simulink model "phase6_regerative"  (R2025a)
settings: Solver=VariableStepAuto  StartTime=0.0  StopTime=5  RelTol=1e-3
model workspace (MAT data in the model file):
  AFE_id_ref_profile = timeseries
  AFE_id_ref_profile.Name = 'unnamed'
  AFE_id_ref_profile.DataInfo = tsdata.datametadata
  AFE_id_ref_profile.DataInfo.Interpolation = tsdata.interpolation
  AFE_id_ref_profile.DataInfo.Interpolation.Fhandle : function handle (value not decoded)
  AFE_id_ref_profile.DataInfo.Interpolation.Name = 'linear'
  AFE_id_ref_profile.TimeInfo = tsdata.timemetadata
  AFE_id_ref_profile.TimeInfo.Length = 6
  AFE_id_ref_profile.TimeInfo.DuplicateTimes = 0
  AFE_id_ref_profile.TimeInfo.Time_ = [0; 0.1; 2; 3; 3.1; 5]
  AFE_id_ref_profile.TimeInfo.Initialized = 1
  AFE_id_ref_profile.QualityInfo = tsdata.qualmetadata
  AFE_id_ref_profile.Data_ = [0.5; 0.5; 0.5; 0.5; -0.5; -0.5]
  G = 10
  Jeq = 0.8325
  Tgravity = 27.25
  eta = 0.9
  g = 9.81
  mc = 500
  mcw = 600
  mp = 200
  r = 0.25
  speed_cmd = timeseries
  speed_cmd.Name = 'unnamed'
  speed_cmd.DataInfo = tsdata.datametadata
  speed_cmd.DataInfo.Interpolation = tsdata.interpolation
  speed_cmd.DataInfo.Interpolation.Fhandle : function handle (value not decoded)
  speed_cmd.DataInfo.Interpolation.Name = 'linear'
  speed_cmd.TimeInfo = tsdata.timemetadata
  speed_cmd.TimeInfo.Length = 6
  speed_cmd.TimeInfo.DuplicateTimes = 0
  speed_cmd.TimeInfo.Time_ = [0; 0.1; 2; 3; 3.01; 5]
  speed_cmd.TimeInfo.Initialized = 1
  speed_cmd.QualityInfo = tsdata.qualmetadata
  speed_cmd.Data_ = [0; 0; 382; 382; 0; 0]
libraries: slpidlib x3, spsUniversalBridgeLib x2, eeGeneralControl x1, spsPLL3phLib x1, eePmsmFieldOrientedControl x1, spsPWMGenerator2LevelLib x1, spsPermanentMagnetSynchronousMachineLib x1, spsSeriesRLCBranchLib x1, spsThreePhaseSeriesRLCBranchLib x1, spsThreePhaseVIMeasurementLib x1, spsThreePhaseSourceLib x1, spsVoltageMeasurementLib x1
settings Model: Creator=kesav  LastModifiedBy=kesav
settings SolverCC: ZeroCrossAlgorithm=Adaptive

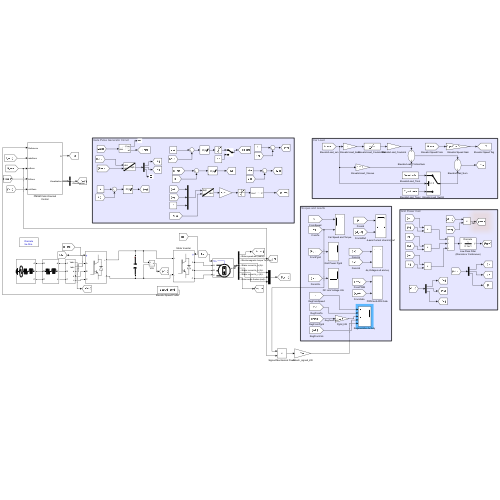
[thumbnail: Simulink's stored preview of the top-level diagram]
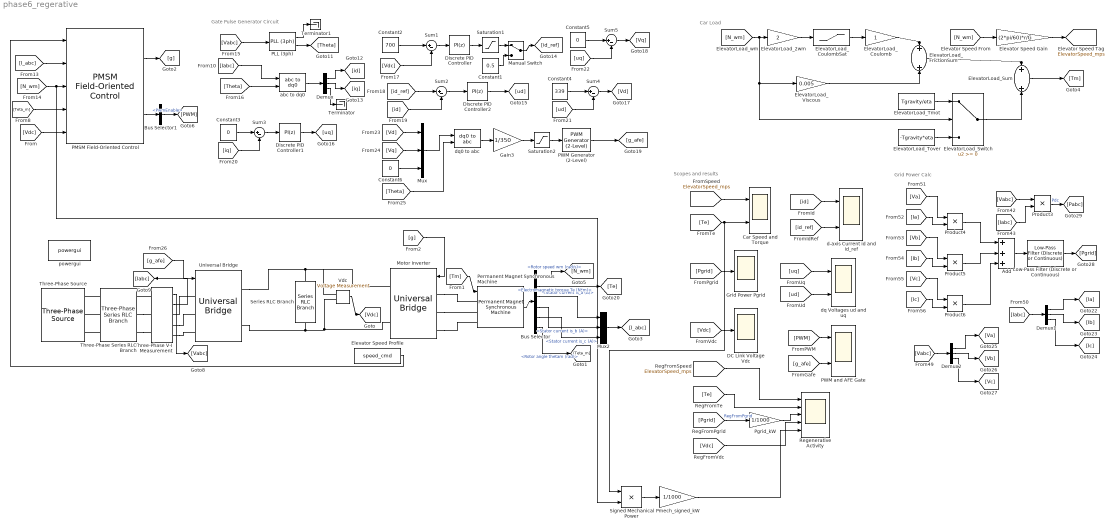
== system phase6_regerative ==
  note: Scopes and results
  note: Grid Power Calc
  note: Car Load
  note: Gate Pulse Generator Circuit
  Add : Sum  Inputs=+++
  Bus Selector : BusSelector  OutputSignals=Rotor speed wm (rad/s),Electromagnetic torque Te (N*m),Stator current is_a (A),Stator current is_b (A),Stator current is_c (A),Rotor angle thetam (rad)
  Bus Selector1 : BusSelector  OutputSignals=PwmEnable
  Car Speed and Torque : Scope  NumInputPorts=2
      settings: ActiveDisplayYMinimum=-0.021018648833083863  ActiveDisplayYMaximum=0.18916306327997173
  Constant1 : Constant  Value=0.5
  Constant2 : Constant  Value=700
  Constant3 : Constant  Value=0
  Constant4 : Constant  Value=339
  Constant5 : Constant  Value=0
  Constant6 : Constant  Value=0
  DC Link Voltage Vdc : Scope
      settings: DataLoggingVariableName=ScopeData2
  Demux : Demux  Outputs=3
  Demux1 : Demux  Outputs=3
  Demux2 : Demux  Outputs=3
  Discrete PID Controller : slpidlib/PID Controller  Controller=PI  Form=Parallel  TimeDomain=Discrete-time  UseExternalTs=off  SampleTime=1e-4  IntegratorMethod=Forward Euler  FilterMethod=Forward Euler  ControllerParametersSource=internal  P=0.5  I=15  UseKiTs=off  D=0  UseExternalDerivativeSource=off  N=100  UseFilter=on  TunerSelectOption=Transfer Function Based (PID Tuner App)  InitialConditionSource=internal  InitialConditionForIntegrator=0  InitialConditionForFilter=0  DifferentiatorICPrevScaledInput=0  ExternalReset=none  TrackingMode=off  Kt=1  LimitOutput=on  SatLimitsSource=internal  UpperSaturationLimit=20  LowerSaturationLimit=-20  LinearizeAsGain=off  AntiWindupMode=clamping  Kb=1  LimitIntegrator=off  UpperIntegratorSaturationLimit=inf  LowerIntegratorSaturationLimit=-inf  POutMin=[]  POutMax=[]  IOutMin=[]  IOutMax=[]  DOutMin=[]  DOutMax=[]  NOutMin=[]  NOutMax=[]  SumOutMin=[]  SumOutMax=[]  SaturationOutMin=[]  SaturationOutMax=[]  PParamMin=[]  PParamMax=[]  IParamMin=[]  IParamMax=[]  DParamMin=[]  DParamMax=[]  NParamMin=[]  NParamMax=[]  KbParamMin=[]  KbParamMax=[]  KtParamMin=[]  KtParamMax=[]  KbOutMin=[]  KbOutMax=[]  KtOutMin=[]  KtOutMax=[]  IntegratorOutMin=[]  IntegratorOutMax=[]  FilterOutMin=[]  FilterOutMax=[]  SumI1OutMin=[]  SumI1OutMax=[]  SumI2OutMin=[]  SumI2OutMax=[]  SumI3OutMin=[]  SumI3OutMax=[]  SumI4OutMin=[]  SumI4OutMax=[]  SumDOutMin=[]  SumDOutMax=[]  DifferentiatorOutMin=[]  DifferentiatorOutMax=[]  FilterDiffOutCoefMin=[]  FilterDiffOutCoefMax=[]  ReciprocalOutMin=[]  ReciprocalOutMax=[]  SumDenOutMin=[]  SumDenOutMax=[]  SumNumOutMin=[]  SumNumOutMax=[]  DivideOutMin=[]  DivideOutMax=[]  UdiffTsProdOutMin=[]  UdiffTsProdOutMax=[]  NTsProdOutMin=[]  NTsProdOutMax=[]  UintegralTsProdOutMin=[]  UintegralTsProdOutMax=[]  UngainTsProdOutMin=[]  UngainTsProdOutMax=[]  ClampingZeroOutDataTypeStr=Inherit: Inherit via back propagation  ClampingZeroOutMin=[]  ClampingZeroOutMax=[]  FilterDenConstantOutDataTypeStr=Inherit: Inherit via back propagation  FilterDenConstantOutMin=[]  FilterDenConstantOutMax=[]  PCopyOutDataTypeStr=Inherit: Inherit via back propagation  PCopyOutMin=[]  PCopyOutMax=[]  NCopyOutDataTypeStr=Inherit: Inherit via back propagation  NCopyOutMin=[]  NCopyOutMax=[]  IntegratorContinuousStateAttributes=''  IntegratorStateMustResolveToSignalObject=off  IntegratorRTWStateStorageClass=Auto  FilterContinuousStateAttributes=''  FilterStateMustResolveToSignalObject=off  FilterRTWStateStorageClass=Auto  ParallelPVariant=InternalParameters  IdealPVariant=Disabled  IVariant=InternalParameters  DVariant=Disabled  IntegratorVariant=Discrete  SatVariant=Enabled  AWVariant=DiscClampingParallel  PCopyVariant=Disabled  TRVariant=Disabled  FdbkBlocksVariant=Forward  IdealPFdbkVariant=Disabled  SatFdbkVariant=Disabled  DerivativeFilterVariant=Disabled  NVariant=Disabled  NCopyVariant=Disabled_SignalSpec  FilterICVariant=Disabled  IntegratorICVariant=InternalICs  ExternalResetVariant=Disabled  TRSumVariant=Passthrough  SumFdbkVariant=Disabled  SumVariant=Sum_PI  TsampFilterVariant=InternalTs  TsampNgainVariant=Passthrough  TsampIntegralVariant=Disabled_SignalSpec  ExternalSaturationOutDataTypeStr=Inherit: Same as second input  DerivativeSourceVariant=Disabled  PreIntVariant=InternalPreInt
      settings: LibrarySourceBlock=simulink/Discrete/Discrete PID Controller
  Discrete PID Controller1 : slpidlib/PID Controller  Controller=PI  Form=Parallel  TimeDomain=Discrete-time  UseExternalTs=off  SampleTime=5e-6  IntegratorMethod=Forward Euler  FilterMethod=Forward Euler  ControllerParametersSource=internal  P=15  I=30  UseKiTs=off  D=0  UseExternalDerivativeSource=off  N=100  UseFilter=on  TunerSelectOption=Transfer Function Based (PID Tuner App)  InitialConditionSource=internal  InitialConditionForIntegrator=0  InitialConditionForFilter=0  DifferentiatorICPrevScaledInput=0  ExternalReset=none  TrackingMode=off  Kt=1  LimitOutput=on  SatLimitsSource=internal  UpperSaturationLimit=350  LowerSaturationLimit=-350  LinearizeAsGain=off  AntiWindupMode=clamping  Kb=1  LimitIntegrator=off  UpperIntegratorSaturationLimit=inf  LowerIntegratorSaturationLimit=-inf  POutMin=[]  POutMax=[]  IOutMin=[]  IOutMax=[]  DOutMin=[]  DOutMax=[]  NOutMin=[]  NOutMax=[]  SumOutMin=[]  SumOutMax=[]  SaturationOutMin=[]  SaturationOutMax=[]  PParamMin=[]  PParamMax=[]  IParamMin=[]  IParamMax=[]  DParamMin=[]  DParamMax=[]  NParamMin=[]  NParamMax=[]  KbParamMin=[]  KbParamMax=[]  KtParamMin=[]  KtParamMax=[]  KbOutMin=[]  KbOutMax=[]  KtOutMin=[]  KtOutMax=[]  IntegratorOutMin=[]  IntegratorOutMax=[]  FilterOutMin=[]  FilterOutMax=[]  SumI1OutMin=[]  SumI1OutMax=[]  SumI2OutMin=[]  SumI2OutMax=[]  SumI3OutMin=[]  SumI3OutMax=[]  SumI4OutMin=[]  SumI4OutMax=[]  SumDOutMin=[]  SumDOutMax=[]  DifferentiatorOutMin=[]  DifferentiatorOutMax=[]  FilterDiffOutCoefMin=[]  FilterDiffOutCoefMax=[]  ReciprocalOutMin=[]  ReciprocalOutMax=[]  SumDenOutMin=[]  SumDenOutMax=[]  SumNumOutMin=[]  SumNumOutMax=[]  DivideOutMin=[]  DivideOutMax=[]  UdiffTsProdOutMin=[]  UdiffTsProdOutMax=[]  NTsProdOutMin=[]  NTsProdOutMax=[]  UintegralTsProdOutMin=[]  UintegralTsProdOutMax=[]  UngainTsProdOutMin=[]  UngainTsProdOutMax=[]  ClampingZeroOutDataTypeStr=Inherit: Inherit via back propagation  ClampingZeroOutMin=[]  ClampingZeroOutMax=[]  FilterDenConstantOutDataTypeStr=Inherit: Inherit via back propagation  FilterDenConstantOutMin=[]  FilterDenConstantOutMax=[]  PCopyOutDataTypeStr=Inherit: Inherit via back propagation  PCopyOutMin=[]  PCopyOutMax=[]  NCopyOutDataTypeStr=Inherit: Inherit via back propagation  NCopyOutMin=[]  NCopyOutMax=[]  IntegratorContinuousStateAttributes=''  IntegratorStateMustResolveToSignalObject=off  IntegratorRTWStateStorageClass=Auto  FilterContinuousStateAttributes=''  FilterStateMustResolveToSignalObject=off  FilterRTWStateStorageClass=Auto  ParallelPVariant=InternalParameters  IdealPVariant=Disabled  IVariant=InternalParameters  DVariant=Disabled  IntegratorVariant=Discrete  SatVariant=Enabled  AWVariant=DiscClampingParallel  PCopyVariant=Disabled  TRVariant=Disabled  FdbkBlocksVariant=Forward  IdealPFdbkVariant=Disabled  SatFdbkVariant=Disabled  DerivativeFilterVariant=Disabled  NVariant=Disabled  NCopyVariant=Disabled_SignalSpec  FilterICVariant=Disabled  IntegratorICVariant=InternalICs  ExternalResetVariant=Disabled  TRSumVariant=Passthrough  SumFdbkVariant=Disabled  SumVariant=Sum_PI  TsampFilterVariant=InternalTs  TsampNgainVariant=Passthrough  TsampIntegralVariant=Disabled_SignalSpec  ExternalSaturationOutDataTypeStr=Inherit: Same as second input  DerivativeSourceVariant=Disabled  PreIntVariant=InternalPreInt
      settings: LibrarySourceBlock=simulink/Discrete/Discrete PID Controller
  Discrete PID Controller2 : slpidlib/PID Controller  Controller=PI  Form=Parallel  TimeDomain=Discrete-time  UseExternalTs=off  SampleTime=5e-6  IntegratorMethod=Forward Euler  FilterMethod=Forward Euler  ControllerParametersSource=internal  P=15  I=30  UseKiTs=off  D=0  UseExternalDerivativeSource=off  N=100  UseFilter=on  TunerSelectOption=Transfer Function Based (PID Tuner App)  InitialConditionSource=internal  InitialConditionForIntegrator=0  InitialConditionForFilter=0  DifferentiatorICPrevScaledInput=0  ExternalReset=none  TrackingMode=off  Kt=1  LimitOutput=on  SatLimitsSource=internal  UpperSaturationLimit=350  LowerSaturationLimit=-350  LinearizeAsGain=off  AntiWindupMode=clamping  Kb=1  LimitIntegrator=off  UpperIntegratorSaturationLimit=inf  LowerIntegratorSaturationLimit=-inf  POutMin=[]  POutMax=[]  IOutMin=[]  IOutMax=[]  DOutMin=[]  DOutMax=[]  NOutMin=[]  NOutMax=[]  SumOutMin=[]  SumOutMax=[]  SaturationOutMin=[]  SaturationOutMax=[]  PParamMin=[]  PParamMax=[]  IParamMin=[]  IParamMax=[]  DParamMin=[]  DParamMax=[]  NParamMin=[]  NParamMax=[]  KbParamMin=[]  KbParamMax=[]  KtParamMin=[]  KtParamMax=[]  KbOutMin=[]  KbOutMax=[]  KtOutMin=[]  KtOutMax=[]  IntegratorOutMin=[]  IntegratorOutMax=[]  FilterOutMin=[]  FilterOutMax=[]  SumI1OutMin=[]  SumI1OutMax=[]  SumI2OutMin=[]  SumI2OutMax=[]  SumI3OutMin=[]  SumI3OutMax=[]  SumI4OutMin=[]  SumI4OutMax=[]  SumDOutMin=[]  SumDOutMax=[]  DifferentiatorOutMin=[]  DifferentiatorOutMax=[]  FilterDiffOutCoefMin=[]  FilterDiffOutCoefMax=[]  ReciprocalOutMin=[]  ReciprocalOutMax=[]  SumDenOutMin=[]  SumDenOutMax=[]  SumNumOutMin=[]  SumNumOutMax=[]  DivideOutMin=[]  DivideOutMax=[]  UdiffTsProdOutMin=[]  UdiffTsProdOutMax=[]  NTsProdOutMin=[]  NTsProdOutMax=[]  UintegralTsProdOutMin=[]  UintegralTsProdOutMax=[]  UngainTsProdOutMin=[]  UngainTsProdOutMax=[]  ClampingZeroOutDataTypeStr=Inherit: Inherit via back propagation  ClampingZeroOutMin=[]  ClampingZeroOutMax=[]  FilterDenConstantOutDataTypeStr=Inherit: Inherit via back propagation  FilterDenConstantOutMin=[]  FilterDenConstantOutMax=[]  PCopyOutDataTypeStr=Inherit: Inherit via back propagation  PCopyOutMin=[]  PCopyOutMax=[]  NCopyOutDataTypeStr=Inherit: Inherit via back propagation  NCopyOutMin=[]  NCopyOutMax=[]  IntegratorContinuousStateAttributes=''  IntegratorStateMustResolveToSignalObject=off  IntegratorRTWStateStorageClass=Auto  FilterContinuousStateAttributes=''  FilterStateMustResolveToSignalObject=off  FilterRTWStateStorageClass=Auto  ParallelPVariant=InternalParameters  IdealPVariant=Disabled  IVariant=InternalParameters  DVariant=Disabled  IntegratorVariant=Discrete  SatVariant=Enabled  AWVariant=DiscClampingParallel  PCopyVariant=Disabled  TRVariant=Disabled  FdbkBlocksVariant=Forward  IdealPFdbkVariant=Disabled  SatFdbkVariant=Disabled  DerivativeFilterVariant=Disabled  NVariant=Disabled  NCopyVariant=Disabled_SignalSpec  FilterICVariant=Disabled  IntegratorICVariant=InternalICs  ExternalResetVariant=Disabled  TRSumVariant=Passthrough  SumFdbkVariant=Disabled  SumVariant=Sum_PI  TsampFilterVariant=InternalTs  TsampNgainVariant=Passthrough  TsampIntegralVariant=Disabled_SignalSpec  ExternalSaturationOutDataTypeStr=Inherit: Same as second input  DerivativeSourceVariant=Disabled  PreIntVariant=InternalPreInt
      settings: LibrarySourceBlock=simulink/Discrete/Discrete PID Controller
  Elevator Speed Gain : Gain  Gain=(2*pi/60)*r/G
  Elevator Speed Profile : FromWorkspace  VariableName=speed_cmd
  ElevatorLoad_2wm : Gain  Gain=2
  ElevatorLoad_Coulomb : Gain
  ElevatorLoad_CoulombSat : Saturate  UpperLimit=1  LowerLimit=-1
  ElevatorLoad_FrictionSum : Sum
  ElevatorLoad_Sum : Sum
  ElevatorLoad_Switch : Switch  SaturateOnIntegerOverflow=off  InputSameDT=off
  ElevatorLoad_Tmot : Constant  Value=Tgravity/eta
  ElevatorLoad_Tover : Constant  Value=-Tgravity*eta
  ElevatorLoad_Viscous : Gain  Gain=0.005
  Gain3 : Gain  Gain=1/350
  Grid Power Pgrid : Scope
      settings: DataLoggingVariableName=ScopeData3
  Low-Pass Filter (Discrete or Continuous) : eeGeneralControl/Low-Pass Filter (Discrete or Continuous)  K=1  T=0.1  B=inf  A=-inf  init_option=Inherited from block input  x0=0  Ts=-1
  Manual Switch : ManualSwitch
  Motor Inverter : spsUniversalBridgeLib/Universal Bridge  Arms=3  SnubberResistance=1e5  SnubberCapacitance=inf  Device=IGBT / Diodes  Ron=1e-3  Lon=0  ForwardVoltages="[  0  0  ]"  ForwardVoltage=0  GTOparameters=[ 10e-6 , 20e-6 ]  IGBTparameters=[ 1e-6 , 2e-6 ]  Measurements=None  Measurements_2=None  converterType=Rectifier
  Mux : Mux  Inputs=3
  Mux2 : Mux  Inputs=3
  PLL (3ph) : spsPLL3phLib/PLL (3ph)  Fmin=45  Par_Init=[0, 50]  ParK=[180, 3200, 1]  TcD=1e-4  MaxRateChangeFreq=12  FilterCutOffFreq=25  Ts=1e-4  AGC=on
  PMSM Field-Oriented Control : eePmsmFieldOrientedControl/PMSM Field-Oriented Control  winding_type=Wye-wound  CtrlMode=Velocity control  Vnom=560  Pmax=75000  Tmax=40  p=4  Vdc_on=100  Ts=5e-6  Tsc=1e-4  CtrlType=PI control  Kp_w=15  Ki_w=50  Kv_w=1  Kaw_w=10  RefType=Zero d-axis control  rpmVec=[0, 3000]  TqVec=[-100, 0, 100]  VdcVec=[300, 350]  PWMMode=SVM: space vector modulation  ModFactor=1  idMatrix=zeros(2,3,2)  iqMatrix=zeros(2,3,2)  psim=0.1194  Ld=0.00024  Lq=0.00029  Rs=0.01  AxisAlignment=D-axis  Kp_id=0.745  Ki_id=91  Kaw_id=1  Kp_iq=0.745  Ki_iq=91  Kaw_iq=1  AxisPrio=Q-axis  ActZC=off  ActFF=on  ParamTypeFF=Constant parameters  LdFF=0.000395  LqFF=0.000395  psimFF=0.1194  idVect=[-200, 0, 200]  iqVect=[-200, 0, 200]  LdMatrix=0.0002 * ones(3, 3)  LqMatrix=0.0002 * ones(3, 3)  psimMatrix=0.04 * ones(3, 3)  CPWMMode=SVM: space vector modulation  fsw=1000
      settings: LibrarySourceBlock=|
      | ee_sl_lib/PMSM Control/PMSM Field-Oriented
      | Control
  PWM Generator (2-Level) : spsPWMGenerator2LevelLib/PWM Generator (2-Level)  ModulatorType=Three-phase bridge (6 pulses)  ModulatorMode=Unsynchronized  Fc=27*60  Pc=90  nF=27  MinMax="[ -1  1 ]"  SamplingTechnique=Natural  ModulatingSignals=off  m=0.8  Freq=60  Phase=0  Ts=0  ShowCarrierOutport=off
  PWM and AFE Gate : Scope  NumInputPorts=2
      settings: DataLoggingVariableName=ScopeData4
  Permanent Magnet Synchronous Machine : spsPermanentMagnetSynchronousMachineLib/Permanent Magnet Synchronous Machine  NbPhases=3  FluxDistribution=Sinusoidal  RotorType=Round  MechanicalLoad=Torque Tm  PresetModel=No  ShowDetailedParameters=on  MeasurementBus=off  Resistance=0.5  Inductance=8.5e-3  dqInductances=[8.5e-3,8.5e-3]  La=7e-3  MachineConstant=Flux linkage established by magnets (V.s)  Flux=0.1194  VoltageCst=86.6271  TorqueCst=0.7164  Flat=120  Mechanical=[Jeq 0.0004924 4 0]  PolePairs=4  InitialConditions=[0,0, 0,0]  InitialConditions5ph=[0 0 0 0 0 0]  RefAngle=Aligned with phase A axis (original Park)  IterativeDiscreteModel=Trapezoidal non iterative  TsBlock=-1  TsPowergui=0
  Pgrid_kW : Gain  Gain=1/1000
  Pmech_signed_kW : Gain  Gain=1/1000
  Product{3..6} (4 alike) : Product
  Regenerative Activity : Scope  NumInputPorts=5
      settings: ActiveDisplayYMinimum=-0.021018648833083863  ActiveDisplayYMaximum=0.18916306327997173  DataLoggingVariableName=regenScopeData
  Saturation1 : Saturate  UpperLimit=20  LowerLimit=-20
  Saturation2 : Saturate  UpperLimit=1  LowerLimit=-1
  Series RLC Branch : spsSeriesRLCBranchLib/Series RLC Branch  LConnTagsString=__new0  RConnTagsString=__new0  BranchType=C  Resistance=0.01  Inductance=1e-3  SetiL0=off  InitialCurrent=0  Capacitance=3e-3  Setx0=on  InitialVoltage=587  Measurements=None
  Signed Mechanical Power : Product  Inputs=**
  Sum{1..5} (5 alike) : Sum  Inputs=|+-
  Terminator : Terminator
  Terminator1 : Terminator
  Three-Phase Series RLC Branch : spsThreePhaseSeriesRLCBranchLib/Three-Phase Series RLC Branch  LConnTagsString=A|B|C  RConnTagsString=A|B|C  BranchType=RL  Resistance=0.5  Inductance=5e-3  Capacitance=1e-6  Measurements=None
  Three-Phase V-I Measurement : spsThreePhaseVIMeasurementLib/Three-Phase V-I Measurement  VoltageMeasurement=phase-to-ground  SetLabelV=off  LabelV=Vabc  Vpu=off  VpuLL=off  CurrentMeasurement=yes  SetLabelI=off  LabelI=Iabc  Ipu=off  Pbase=100e6  Vbase=500e3  OutputType=Complex  PhasorSimulation=off  PSBequivalent=0
  Three-Phase Source : spsThreePhaseSourceLib/Three-Phase Source  InternalConnection=Yg  VoltagePhases=off  Voltage=415  PhaseAngle=0  Voltage_phases=[25e3 25e3 25e3]/sqrt(3)  PhaseAngles_phases=[0 -120 +120]  Frequency=50  NonIdealSource=on  SpecifyImpedance=off  Resistance=0.05  Inductance=0.5e-3  ShortCircuitLevel=100e6  BaseVoltage=25e3  XRratio=7  BusType=swing  Pref=10e3  Qref=0  Prefabc=[10e3, 10e3, 10e3]  Qrefabc=[0, 0, 0]  Qmin=-inf  Qmax=inf
  Universal Bridge : spsUniversalBridgeLib/Universal Bridge  Arms=3  SnubberResistance=1e5  SnubberCapacitance=inf  Device=IGBT / Diodes  Ron=1e-3  Lon=0  ForwardVoltages="[  0  0  ]"  ForwardVoltage=0  GTOparameters=[ 10e-6 , 20e-6 ]  IGBTparameters=[ 1e-6 , 2e-6 ]  Measurements=None  Measurements_2=None  converterType=Rectifier
  Vdc : spsVoltageMeasurementLib/Voltage Measurement  PhasorSimulation=off  OutputType=Complex  PSBequivalent=0
  abc to dq0 : spsabctodq0Lib/abc to dq0  Alignment=90 degrees behind phase A axis
  d-axis Current id and id_ref : Scope  NumInputPorts=2
      settings: ActiveDisplayYMinimum=-9.75848157655837  ActiveDisplayYMaximum=32.389133382764612  DataLoggingVariableName=ScopeData5
  dq Voltages ud and uq : Scope  NumInputPorts=2
  dq0 to abc : spsdq0toabcLib/dq0 to abc  Alignment=90 degrees behind phase A axis
  powergui : spspowerguiLib/powergui  Priority=1  SimulationMode=Discrete  SampleTime=5e-6  frequency=60  Iterations=50  frequencyindice=0  Pbase=100e6  ErrMax=1e-4  UnitsV=kV  UnitsW=MW  buscounter=0  FunctionMessages=off  echomessages=off  EnableUseOfTLC=off  CurrentSourceSwitches=off  DisableSnubberDevices=off  DisableRonSwitches=off  DisableVfSwitches=off  DisplayEquations=off  AutomaticDiscreteSolvers=off  SolverType=Tustin/Backward Euler (TBE)  Interpol=off  ExternalGateDelay=off  methode=off  Ts=100  x0status=blocks  SPID=on  SwTol=0  HookPort=off  NonlinearTolerance=1e-4  nMaxIteration=100  ContinueOnMaxIteration=off  RestoreLinks=warning  ResistiveCurrentMeasurement=off  Frange=[0:2:500]  Ylog=off  Xlog=on  ShowGrid=off  save=off  variable=ZData  structure=0  ZoomFFT=off  StartTime=0.0  cycles=1  DisplayStyle=1  fundamental=60  FreqAxis=off  MaxFrequency=1000  frequencyindicesteady=1  RmsSteady=1  display=off
  tag scope: ElevatorSpeed_mps=global
  wires:
  Vdc/1 -> [Vdc]
  Permanent Magnet Synchronous Machine/1 -> Bus Selector/1
  [g] -> Motor Inverter/1
  Bus Selector/6 -> [Teta_m]  "<Rotor angle thetam (rad)>"
  Bus Selector/3 -> Mux2/1  "<Stator current is_a (A)>"
  Mux2/1 -> [I_abc]
  Bus Selector/4 -> Mux2/2  "<Stator current is_b (A)>"
  Bus Selector/5 -> Mux2/3  "<Stator current is_c (A)>"
  Bus Selector/1 -> [N_wm]  "<Rotor speed wm (rad/s)>"
  [I_abc] -> PMSM Field-Oriented Control/2
  [N_wm] -> PMSM Field-Oriented Control/3, Signed Mechanical Power/2
  [Vdc] -> PMSM Field-Oriented Control/5
  PMSM Field-Oriented Control/2 -> Bus Selector1/1
  PMSM Field-Oriented Control/1 -> [g]
  Bus Selector1/1 -> [PWM]  "<PwmEnable>"
  [Teta_m] -> PMSM Field-Oriented Control/4
  Three-Phase V-I Measurement/1 -> [Vabc]
  Three-Phase V-I Measurement/2 -> [Iabc]
  [Vabc] -> PLL (3ph)/1
  PLL (3ph)/2 -> [Theta]
  [Theta] -> abc to dq0/2
  [Iabc] -> abc to dq0/1
  abc to dq0/1 -> Demux/1
  Demux/1 -> [id]
  Demux/2 -> [iq]
  Constant2/1 -> Sum1/1
  [Vdc] -> Sum1/2
  Sum1/1 -> Discrete PID Controller/1
  Discrete PID Controller/1 -> Saturation1/1
  [id_ref] -> Sum2/1
  [id] -> Sum2/2
  Sum2/1 -> Discrete PID Controller2/1
  Discrete PID Controller2/1 -> [ud]
  Sum3/1 -> Discrete PID Controller1/1
  Discrete PID Controller1/1 -> [uq]
  [iq] -> Sum3/2
  Constant3/1 -> Sum3/1
  PLL (3ph)/1 -> Terminator1/1
  Demux/3 -> Terminator/1
  Constant4/1 -> Sum4/1
  [ud] -> Sum4/2
  Sum4/1 -> [Vd]
  Sum5/1 -> [Vq]
  [uq] -> Sum5/2
  Constant5/1 -> Sum5/1
  [Vd] -> Mux/1
  [Vq] -> Mux/2
  Constant6/1 -> Mux/3
  Mux/1 -> dq0 to abc/1
  [Theta] -> dq0 to abc/2
  dq0 to abc/1 -> Gain3/1
  Gain3/1 -> Saturation2/1
  Saturation2/1 -> PWM Generator (2-Level)/1
  PWM Generator (2-Level)/1 -> [g_afe]
  [g_afe] -> Universal Bridge/1
  Bus Selector/2 -> [Te]  "<Electromagnetic torque Te (N*m)>"
  [Vabc] -> Product3/1
  [Iabc] -> Product3/2
  [Iabc] -> Demux1/1
  Demux1/1 -> [Ia]
  Demux1/2 -> [Ib]
  Demux1/3 -> [Ic]
  Demux2/1 -> [Va]
  Demux2/3 -> [Vc]
  Demux2/2 -> [Vb]
  [Vabc] -> Demux2/1
  [Va] -> Product4/1
  [Ia] -> Product4/2
  [Ib] -> Product5/2
  [Vb] -> Product5/1
  [Ic] -> Product6/2
  [Vc] -> Product6/1
  Product4/1 -> Add/1
  Product5/1 -> Add/2
  Product6/1 -> Add/3
  Add/1 -> Low-Pass Filter (Discrete or Continuous)/1
  Low-Pass Filter (Discrete or Continuous)/1 -> [Pgrid]
  Product3/1 -> [Pabc]  "Pdc"
  Saturation1/1 -> Manual Switch/1
  Constant1/1 -> Manual Switch/2
  [N_wm] -> Elevator Speed Gain/1
  Elevator Speed Gain/1 -> [ElevatorSpeed_mps]
  [g_afe] -> PWM and AFE Gate/2
  [PWM] -> PWM and AFE Gate/1
  [ud] -> dq Voltages ud and uq/2
  [uq] -> dq Voltages ud and uq/1
  [Pgrid] -> Grid Power Pgrid/1
  [id] -> d-axis Current id and id_ref/1
  [id_ref] -> d-axis Current id and id_ref/2
  [Vdc] -> DC Link Voltage Vdc/1
  [ElevatorSpeed_mps] -> Regenerative Activity/1
  [Te] -> Regenerative Activity/2
  [Pgrid] -> Pgrid_kW/1  "RegFromPgrid"
  [Vdc] -> Regenerative Activity/4
  Pgrid_kW/1 -> Regenerative Activity/3
  [N_wm] -> ElevatorLoad_Viscous/1, ElevatorLoad_Switch/2, ElevatorLoad_2wm/1
  ElevatorLoad_2wm/1 -> ElevatorLoad_CoulombSat/1
  ElevatorLoad_CoulombSat/1 -> ElevatorLoad_Coulomb/1
  ElevatorLoad_Coulomb/1 -> ElevatorLoad_FrictionSum/1
  ElevatorLoad_Viscous/1 -> ElevatorLoad_FrictionSum/2
  ElevatorLoad_Tmot/1 -> ElevatorLoad_Switch/1
  ElevatorLoad_Tover/1 -> ElevatorLoad_Switch/3
  [Tm] -> Permanent Magnet Synchronous Machine/1
  ElevatorLoad_Sum/1 -> [Tm]
  ElevatorLoad_FrictionSum/1 -> ElevatorLoad_Sum/1
  ElevatorLoad_Switch/1 -> ElevatorLoad_Sum/2
  [ElevatorSpeed_mps] -> Car Speed and Torque/1
  [Te] -> Car Speed and Torque/2, Signed Mechanical Power/1
  Elevator Speed Profile/1 -> PMSM Field-Oriented Control/1
  Manual Switch/1 -> [id_ref]
  Signed Mechanical Power/1 -> Pmech_signed_kW/1
  Pmech_signed_kW/1 -> Regenerative Activity/5
  connections:
  Motor Inverter/LConn1 -- Permanent Magnet Synchronous Machine/LConn1
  Motor Inverter/LConn2 -- Permanent Magnet Synchronous Machine/LConn2
  Motor Inverter/LConn3 -- Permanent Magnet Synchronous Machine/LConn3
  Three-Phase Series RLC Branch/LConn1 -- Three-Phase Source/RConn1
  Three-Phase Series RLC Branch/LConn2 -- Three-Phase Source/RConn2
  Three-Phase Series RLC Branch/LConn3 -- Three-Phase Source/RConn3
  Three-Phase V-I Measurement/LConn1 -- Three-Phase Series RLC Branch/RConn1
  Three-Phase Series RLC Branch/RConn2 -- Three-Phase V-I Measurement/LConn2
  Three-Phase Series RLC Branch/RConn3 -- Three-Phase V-I Measurement/LConn3
  Three-Phase V-I Measurement/RConn3 -- Universal Bridge/LConn3
  Three-Phase V-I Measurement/RConn2 -- Universal Bridge/LConn2
  Three-Phase V-I Measurement/RConn1 -- Universal Bridge/LConn1
  Vdc/LConn2 -- Motor Inverter/RConn2 -- Universal Bridge/RConn2 -- Series RLC Branch/RConn1
  Universal Bridge/RConn1 -- Vdc/LConn1 -- Motor Inverter/RConn1 -- Series RLC Branch/LConn1
